simulink model "Boost_Converter_Interleaved"  (R2022a)
settings: Solver=VariableStepAuto  StartTime=0.0  StopTime=1  RelTol=1e-3
libraries: spsSeriesRLCBranchLib x4, spsCurrentMeasurementLib x2, spsDiodeLib x2, spsMosfetLib x2, eePowerMeasurement x2, spsVoltageMeasurementLib x2, spsDCVoltageSourceLib x1, spspowerguiLib x1
settings Model: Creator=Bobby  LastModifiedBy=Bobby

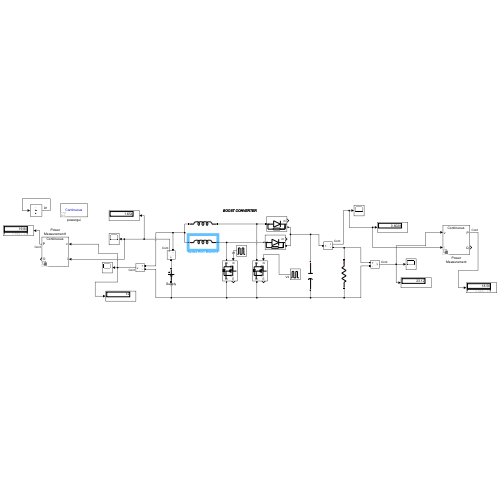
[thumbnail: Simulink's stored preview of the top-level diagram]
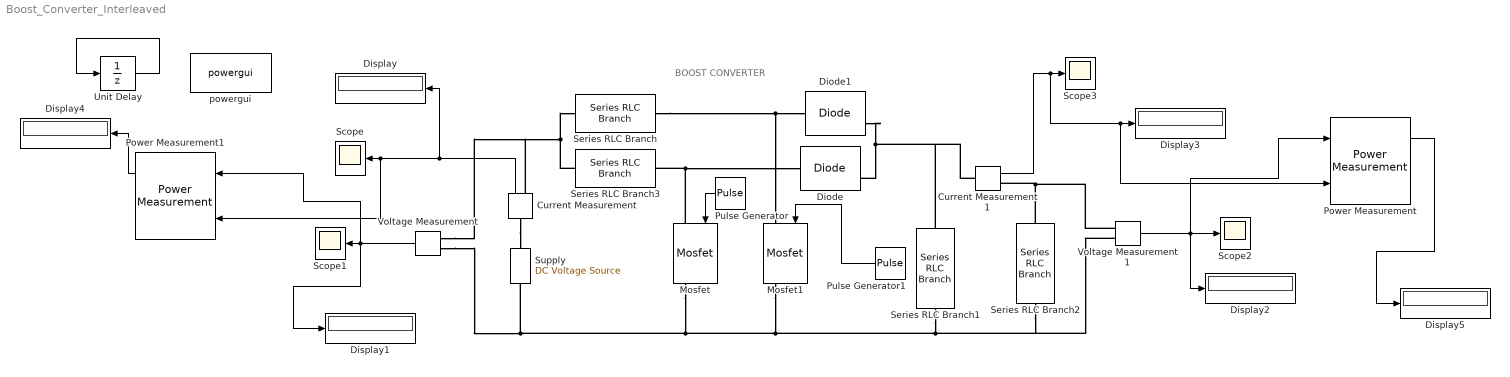
== system Boost_Converter_Interleaved ==
  note: BOOST CONVERTER
  Current Measurement : spsCurrentMeasurementLib/Current Measurement  PhasorSimulation=off  OutputType=Complex  PSBequivalent=0
  Current Measurement1 : spsCurrentMeasurementLib/Current Measurement  PhasorSimulation=off  OutputType=Complex  PSBequivalent=0
  Diode : spsDiodeLib/Diode  Ron=0.001  Lon=0  Vf=0.8  IC=0  UseSnubber=0  Rs=500  Cs=250e-9  Measurements=on
  Diode1 : spsDiodeLib/Diode  Ron=0.001  Lon=0  Vf=0.8  IC=0  UseSnubber=0  Rs=500  Cs=250e-9  Measurements=on
  Display{,1..5} (6 alike) : Display
  Mosfet : spsMosfetLib/Mosfet  Ron=0.1  Lon=0  Rd=0.01  Vfd=0  IC=0  Rs=1e5  Cs=inf  Measurements=on
  Mosfet1 : spsMosfetLib/Mosfet  Ron=0.1  Lon=0  Rd=0.01  Vfd=0  IC=0  Rs=1e5  Cs=inf  Measurements=on
  Power Measurement : eePowerMeasurement/Power Measurement  LabelModeActiveChoice=Continuous  F=60  K=[0 1 2 3]  Ts=0
      settings: SourceProductBaseCode=PS
  Power Measurement1 : eePowerMeasurement/Power Measurement  LabelModeActiveChoice=Continuous  F=60  K=[0 1 2 3]  Ts=0
      settings: SourceProductBaseCode=PS
  Pulse Generator : DiscretePulseGenerator  PulseType=Time based  Period=0.00002  PulseWidth=50
  Pulse Generator1 : DiscretePulseGenerator  PulseType=Time based  Period=0.00002  PulseWidth=50  PhaseDelay=10e-6
  Scope{,1..3} (4 alike) : Scope
  Series RLC Branch : spsSeriesRLCBranchLib/Series RLC Branch  LConnTagsString=__new0  RConnTagsString=__new0  BranchType=L  Resistance=1  Inductance=650e-6  SetiL0=off  InitialCurrent=0  Capacitance=1e-6  Setx0=off  InitialVoltage=0  Measurements=None
  Series RLC Branch1 : spsSeriesRLCBranchLib/Series RLC Branch  LConnTagsString=__new0  RConnTagsString=__new0  BranchType=C  Resistance=1  Inductance=1e-3  SetiL0=off  InitialCurrent=0  Capacitance=34.7e-6  Setx0=off  InitialVoltage=0  Measurements=None
  Series RLC Branch2 : spsSeriesRLCBranchLib/Series RLC Branch  LConnTagsString=__new0  RConnTagsString=__new0  BranchType=R  Resistance=28.8  Inductance=1e-3  SetiL0=off  InitialCurrent=0  Capacitance=1e-6  Setx0=off  InitialVoltage=0  Measurements=None
  Series RLC Branch3 : spsSeriesRLCBranchLib/Series RLC Branch  LConnTagsString=__new0  RConnTagsString=__new0  BranchType=L  Resistance=1  Inductance=650e-6  SetiL0=on  InitialCurrent=0  Capacitance=1e-6  Setx0=off  InitialVoltage=0  Measurements=None
  Supply : spsDCVoltageSourceLib/DC Voltage Source  Amplitude=12  Measurements=None
  Unit Delay : UnitDelay  SampleTime=-1  HasFrameUpgradeWarning=on
  Voltage Measurement : spsVoltageMeasurementLib/Voltage Measurement  PhasorSimulation=off  OutputType=Complex  PSBequivalent=0
  Voltage Measurement1 : spsVoltageMeasurementLib/Voltage Measurement  PhasorSimulation=off  OutputType=Complex  PSBequivalent=0
  powergui : spspowerguiLib/powergui  Priority=1  SimulationMode=Continuous  SampleTime=50e-6  frequency=60  Iterations=50  frequencyindice=0  Pbase=100e6  ErrMax=1e-4  UnitsV=kV  UnitsW=MW  buscounter=0  FunctionMessages=off  echomessages=off  EnableUseOfTLC=off  CurrentSourceSwitches=off  DisableSnubberDevices=off  DisableRonSwitches=off  DisableVfSwitches=off  DisplayEquations=off  AutomaticDiscreteSolvers=off  SolverType=Tustin/Backward Euler (TBE)  Interpol=off  ExternalGateDelay=off  methode=off  Ts=100  x0status=blocks  SPID=on  SwTol=0  HookPort=off  NonlinearTolerance=1e-4  nMaxIteration=100  ContinueOnMaxIteration=off  RestoreLinks=warning  ResistiveCurrentMeasurement=off  Frange=[0:2:500]  Ylog=off  Xlog=on  ShowGrid=off  save=off  variable=ZData  structure=0  ZoomFFT=off  StartTime=0.0  cycles=1  DisplayStyle=1  fundamental=60  FreqAxis=off  MaxFrequency=1000  frequencyindicesteady=1  RmsSteady=1  display=off
  wires:
  Unit Delay/1 -> Unit Delay/1
  Pulse Generator/1 -> Mosfet/1
  Voltage Measurement/1 -> Display1/1, Scope1/1, Power Measurement1/1
  Current Measurement1/1 -> Power Measurement/2, Display3/1, Scope3/1
  Voltage Measurement1/1 -> Display2/1, Scope2/1, Power Measurement/1
  Current Measurement/1 -> Display/1, Power Measurement1/2, Scope/1
  Pulse Generator1/1 -> Mosfet1/1
  Power Measurement1/1 -> Display4/1
  Power Measurement/1 -> Display5/1
  connections:
  Mosfet/LConn1 -- Diode/LConn1 -- Series RLC Branch3/RConn1
  Mosfet/RConn1 -- Mosfet1/RConn1 -- Series RLC Branch2/RConn1 -- Voltage Measurement1/LConn2 -- Series RLC Branch1/RConn1 -- Voltage Measurement/LConn2 -- Supply/LConn1
  Series RLC Branch2/LConn1 -- Voltage Measurement1/LConn1 -- Current Measurement1/RConn1
  Current Measurement/LConn1 -- Supply/RConn1
  Series RLC Branch3/LConn1 -- Voltage Measurement/LConn1 -- Current Measurement/RConn1 -- Series RLC Branch/LConn1
  Series RLC Branch/RConn1 -- Diode1/LConn1 -- Mosfet1/LConn1
  Diode1/RConn1 -- Series RLC Branch1/LConn1 -- Current Measurement1/LConn1 -- Diode/RConn1
